simulink model "Intelligent_BMS_4S_LiFePO4"  (R2026b)
settings: Solver=FixedStepDiscrete  StopTime=3600  FixedStep=1
undefined symbols (not defined in the file): DiscIntNeverNeededParam
settings Model: Creator=josab  LastModifiedBy=josab

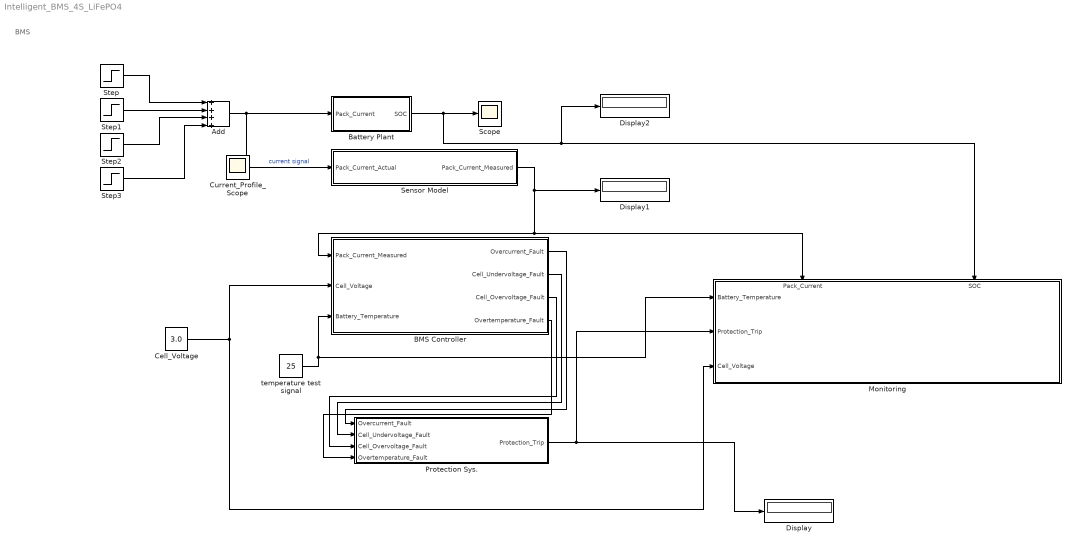
== system Intelligent_BMS_4S_LiFePO4 ==
  note: BMS
  "  Monitoring" : Subsystem
      settings: PortSchema="{\"entries\":[{\"content\":{\"sides\":[{\"content\":{\"connectorIds\":[\"In1\",\"In2\",\"In3\"]},\"type\":\"ConnectorPlacement.EquallySpacedRectSide\",\"uuid\":\"0d678bb2-c0a0-4749-bc78-1b1470b37621\"},{\"content\":{\"side\":\"RIGHT\"},\"type\":\"ConnectorPlacement.EquallySpacedRectSide\",\"uuid\":\"65c4c7ed-0cbd-4dbc-8d8d-31b797dd0dbb\"},{\"content\":{\"connectorIds\":[\"In4\",\"In5\"],\"side\":\"TOP\"},\"type\":\"ConnectorPlacement.EquallySpacedRectSide\",\"uuid\":\"d9b849b5-be61-47a7-987a-fbb34be0c968\"}]},\"type\":\"ConnectorPlacement.EquallySpacedConnector\",\"uuid\":\"8fa5f423-d5fa-40b0-8d3e-a111cf29ff43\"}],\"packageUris\":[\"http://schema.mathworks.com/mf0/Connector/R2020b\"],\"version\":\"1.0\"}"
  "  Sensor Model " : Subsystem
  " BMS Controller " : Subsystem
  Add : Sum  Inputs=++++
  Battery Plant : Subsystem
  Cell_Voltage : Constant  Value=3.0
  Current_Profile_Scope : Scope
      settings: ActiveDisplayYMinimum=4.8052017355806633  ActiveDisplayYMaximum=4.9695325733967586
  Display : Display
  Display1 : Display
  Display2 : Display
  Protection Sys. : Subsystem
  Scope : Scope
      settings: ActiveDisplayYMinimum=0.62939996840347556  ActiveDisplayYMaximum=0.86630316972526478
  Step : Step  Time=0  SampleTime=0
  Step1 : Step  Time=500  FinalValue=2  SampleTime=0
  Step2 : Step  Time=1000  FinalValue=2  SampleTime=0
  Step3 : Step  Time=1500  FinalValue=-3  SampleTime=0
  temperature test signal : Constant  Value=25
  wires:
  Battery Plant/1(SOC) -> Display2/1, "  Monitoring"/5(SOC), Scope/1
  Step/1 -> Add/1
  Step1/1 -> Add/2
  Step2/1 -> Add/3
  Step3/1 -> Add/4
  Add/1 -> "  Sensor Model "/1(Pack_Current_Actual), Current_Profile_Scope/1, Battery Plant/1(Pack_Current)  "current signal"
  "  Sensor Model "/1(Pack_Current_Measured) -> Display1/1, "  Monitoring"/4(Pack_Current), " BMS Controller "/1(Pack_Current_Measured)
  Protection Sys./1(Protection_Trip) -> Display/1, "  Monitoring"/2(Protection_Trip)
  temperature test signal/1 -> "  Monitoring"/1(Battery_Temperature), " BMS Controller "/3(Battery_Temperature)
  " BMS Controller "/1(Overcurrent_Fault) -> Protection Sys./1(Overcurrent_Fault)
  " BMS Controller "/2(Cell_Undervoltage_Fault) -> Protection Sys./2(Cell_Undervoltage_Fault)
  " BMS Controller "/3(Cell_Overvoltage_Fault) -> Protection Sys./3(Cell_Overvoltage_Fault)
  " BMS Controller "/4(Overtemperature_Fault) -> Protection Sys./4(Overtemperature_Fault)
  Cell_Voltage/1 -> "  Monitoring"/3(Cell_Voltage), " BMS Controller "/2(Cell_Voltage)

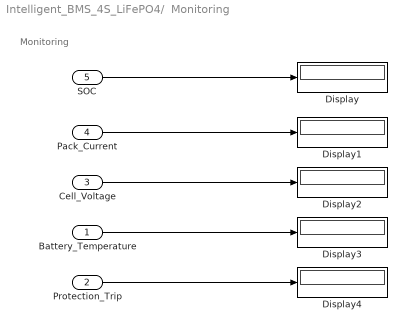
== system Intelligent_BMS_4S_LiFePO4/  Monitoring ==
  note: Monitoring
  Battery_Temperature : Inport
  Protection_Trip : Inport  Port=2
  Cell_Voltage : Inport  Port=3
  Pack_Current : Inport  Port=4
  SOC : Inport  Port=5
  Display{,1..4} (5 alike) : Display
  wires:
  SOC/1 -> Display/1
  Pack_Current/1 -> Display1/1
  Cell_Voltage/1 -> Display2/1
  Battery_Temperature/1 -> Display3/1
  Protection_Trip/1 -> Display4/1

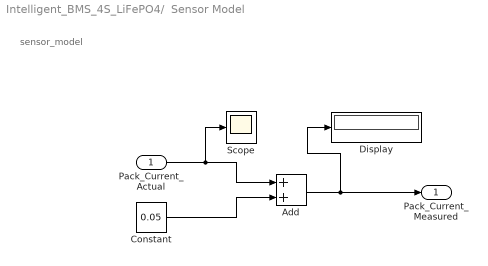
== system Intelligent_BMS_4S_LiFePO4/  Sensor Model  ==
  note: sensor_model
  Pack_Current_Actual : Inport
  Add : Sum
  Constant : Constant  Value=0.05
  Display : Display
  Scope : Scope
      settings: ActiveDisplayYMinimum=0.50000000000000011  ActiveDisplayYMaximum=5.5  DataLoggingVariableName=ScopeData2
  Pack_Current_Measured : Outport
  wires:
  Pack_Current_Actual/1 -> Scope/1, Add/1
  Constant/1 -> Add/2
  Add/1 -> Display/1, Pack_Current_Measured/1

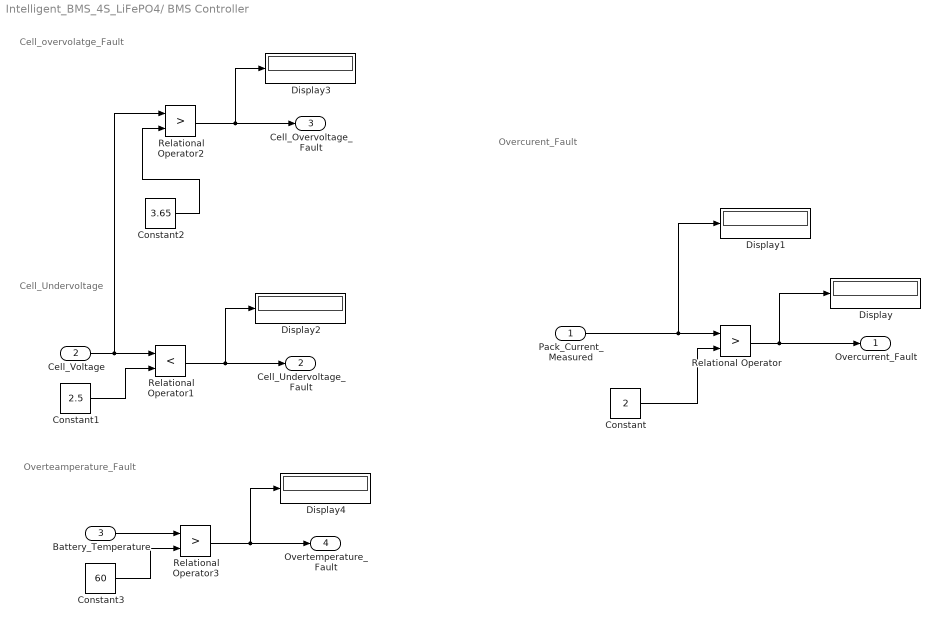
== system Intelligent_BMS_4S_LiFePO4/ BMS Controller  ==
  note: Overteamperature_Fault
  note: Cell_overvolatge_Fault
  note: Cell_Undervoltage
  note: Overcurent_Fault
  Pack_Current_Measured : Inport
  Cell_Voltage : Inport  Port=2
  Battery_Temperature : Inport  Port=3
  Constant : Constant  Value=2
  Constant1 : Constant  Value=2.5
  Constant2 : Constant  Value=3.65
  Constant3 : Constant  Value=60
  Display{,1..4} (5 alike) : Display
  Relational Operator : RelationalOperator  Operator=>  OutDataTypeStr=boolean  RndMeth=Simplest  InputSameDT=off
  Relational Operator1 : RelationalOperator  Operator=<  OutDataTypeStr=boolean  RndMeth=Simplest  InputSameDT=off
  Relational Operator2 : RelationalOperator  Operator=>  OutDataTypeStr=boolean  RndMeth=Simplest  InputSameDT=off
  Relational Operator3 : RelationalOperator  Operator=>  OutDataTypeStr=boolean  RndMeth=Simplest  InputSameDT=off
  Overcurrent_Fault : Outport
  Cell_Undervoltage_Fault : Outport  Port=2
  Cell_Overvoltage_Fault : Outport  Port=3
  Overtemperature_Fault : Outport  Port=4
  wires:
  Pack_Current_Measured/1 -> Display1/1, Relational Operator/1
  Constant/1 -> Relational Operator/2
  Relational Operator/1 -> Display/1, Overcurrent_Fault/1
  Constant1/1 -> Relational Operator1/2
  Relational Operator1/1 -> Display2/1, Cell_Undervoltage_Fault/1
  Cell_Voltage/1 -> Relational Operator1/1, Relational Operator2/1
  Constant2/1 -> Relational Operator2/2
  Relational Operator2/1 -> Display3/1, Cell_Overvoltage_Fault/1
  Battery_Temperature/1 -> Relational Operator3/1
  Constant3/1 -> Relational Operator3/2
  Relational Operator3/1 -> Display4/1, Overtemperature_Fault/1

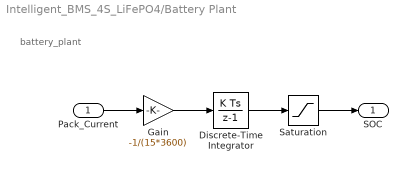
== system Intelligent_BMS_4S_LiFePO4/Battery Plant ==
  note: battery_plant
  Pack_Current : Inport
  Discrete-Time Integrator : DiscreteIntegrator  gainval=1  InitialCondition=0.8  ICPrevOutput=DiscIntNeverNeededParam  ICPrevScaledInput=DiscIntNeverNeededParam
  Gain : Gain  Gain=-1/(15*3600)
  Saturation : Saturate  UpperLimit=1  LowerLimit=0
  SOC : Outport
  wires:
  Pack_Current/1 -> Gain/1
  Gain/1 -> Discrete-Time Integrator/1
  Discrete-Time Integrator/1 -> Saturation/1
  Saturation/1 -> SOC/1

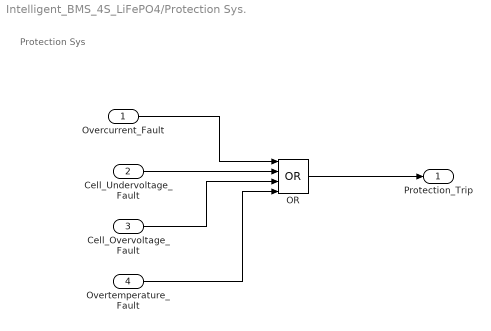
== system Intelligent_BMS_4S_LiFePO4/Protection Sys. ==
  note: Protection Sys
  Overcurrent_Fault : Inport
  Cell_Undervoltage_Fault : Inport  Port=2
  Cell_Overvoltage_Fault : Inport  Port=3
  Overtemperature_Fault : Inport  Port=4
  OR : Logic  Operator=OR  Inputs=4  IconShape=distinctive  AllPortsSameDT=off  OutDataTypeStr=boolean
  Protection_Trip : Outport
  wires:
  Overcurrent_Fault/1 -> OR/1
  Cell_Undervoltage_Fault/1 -> OR/2
  Cell_Overvoltage_Fault/1 -> OR/3
  Overtemperature_Fault/1 -> OR/4
  OR/1 -> Protection_Trip/1
